simulink model "hdlcoder_counters_eml"  (R2026a)
settings: Solver=FixedStepDiscrete  StopTime=15  FixedStep=1
settings Model: Creator=The MathWorks, Inc.  LastModifiedBy=The MathWorks, Inc.
settings OptimizationCC: ConditionallyExecuteInputs=off  InitFltsAndDblsToZero=on
settings DebuggingCC: AlgebraicLoopMsg=error  SaveWithParameterizedLinksMsg=none  UnderspecifiedInitializationDetection=Classic  MultiTaskDSMMsg=warning  MultiTaskCondExecSysMsg=none  SingleTaskRateTransMsg=error
settings HardwareCC: ProdHWDeviceType=Specified
settings GRTTargetCC: TargetFcnLib=ansi_tfl_tmw.mat  CombineOutputUpdateFcns=off  GRTInterface=on

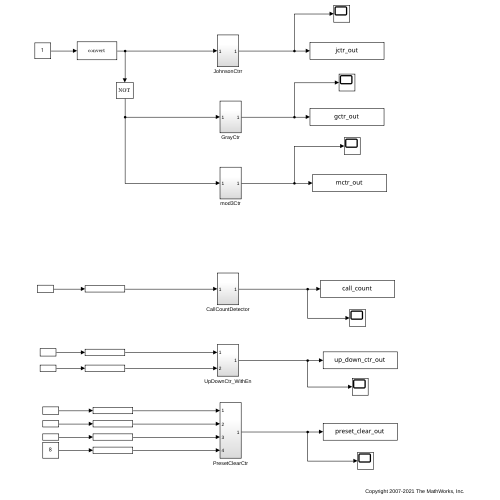
[thumbnail: Simulink's stored preview of the top-level diagram]
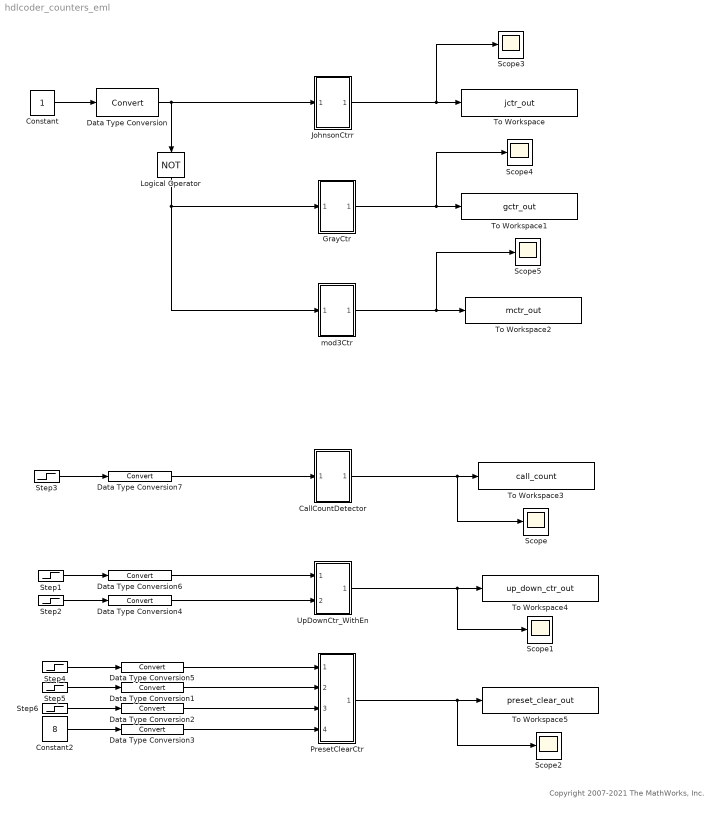
== system hdlcoder_counters_eml ==
  note: Copyright 2007-2021 The MathWorks, Inc.
  CallCountDetector : Subsystem
  Constant : Constant  SampleTime=1
  Constant2 : Constant  Value=8  SampleTime=1
  Data Type Conversion{,1..7} (8 alike) : DataTypeConversion  SaturateOnIntegerOverflow=off  RndMeth=Floor
  GrayCtr : Subsystem
  JohnsonCtrr : Subsystem
  Logical Operator : Logic  Operator=NOT  AllPortsSameDT=off  OutDataTypeStr=boolean
  PresetClearCtr : Subsystem
  Scope{,1..5} (6 alike) : Scope
      Scope2 settings: DataLoggingVariableName=ScopeData2
      Scope3 settings: DataLoggingVariableName=ScopeData3
      Scope4 settings: DataLoggingVariableName=ScopeData4
      Scope5 settings: DataLoggingVariableName=ScopeData5
  Step1 : Step  Time=3  SampleTime=1
  Step2 : Step  Time=7  SampleTime=1
  Step3 : Step  Time=3  SampleTime=1
  Step4 : Step  Time=7  SampleTime=1
  Step5 : Step  Time=2  SampleTime=1
  Step6 : Step  Time=4  SampleTime=1
  To Workspace : ToWorkspace  VariableName=jctr_out  SampleTime=-1
  To Workspace1 : ToWorkspace  VariableName=gctr_out  SampleTime=-1
  To Workspace2 : ToWorkspace  VariableName=mctr_out  SampleTime=-1
  To Workspace3 : ToWorkspace  VariableName=call_count  SampleTime=-1
  To Workspace4 : ToWorkspace  VariableName=up_down_ctr_out  SampleTime=-1
  To Workspace5 : ToWorkspace  VariableName=preset_clear_out  SampleTime=-1
  UpDownCtr_WithEn : Subsystem
  mod3Ctr : Subsystem
  wires:
  Constant/1 -> Data Type Conversion/1
  Data Type Conversion/1 -> Logical Operator/1, JohnsonCtrr/1(In1)
  Logical Operator/1 -> GrayCtr/1(In1), mod3Ctr/1(In1)
  JohnsonCtrr/1(Out1) -> To Workspace/1, Scope3/1
  GrayCtr/1(Out1) -> To Workspace1/1, Scope4/1
  mod3Ctr/1(Out1) -> To Workspace2/1, Scope5/1
  Step4/1 -> Data Type Conversion5/1
  Step5/1 -> Data Type Conversion1/1
  Step6/1 -> Data Type Conversion2/1
  Constant2/1 -> Data Type Conversion3/1
  Data Type Conversion5/1 -> PresetClearCtr/1(In1)
  Data Type Conversion1/1 -> PresetClearCtr/2(In2)
  Data Type Conversion2/1 -> PresetClearCtr/3(In3)
  Data Type Conversion3/1 -> PresetClearCtr/4(In4)
  CallCountDetector/1(Out1) -> To Workspace3/1, Scope/1
  UpDownCtr_WithEn/1(Out1) -> To Workspace4/1, Scope1/1
  PresetClearCtr/1(Out1) -> To Workspace5/1, Scope2/1
  Step1/1 -> Data Type Conversion6/1
  Step2/1 -> Data Type Conversion4/1
  Data Type Conversion6/1 -> UpDownCtr_WithEn/1(In1)
  Data Type Conversion4/1 -> UpDownCtr_WithEn/2(In2)
  Step3/1 -> Data Type Conversion7/1
  Data Type Conversion7/1 -> CallCountDetector/1(In1)

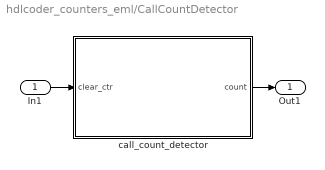
== system hdlcoder_counters_eml/CallCountDetector ==
  In1 : Inport
  call_count_detector : MATLAB Function  TreatAsAtomicUnit=on
  Out1 : Outport
  wires:
  In1/1 -> call_count_detector/1(clear_ctr)
  call_count_detector/1(count) -> Out1/1

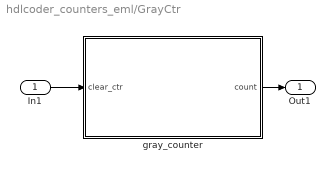
== system hdlcoder_counters_eml/GrayCtr ==
  In1 : Inport
  gray_counter : MATLAB Function  TreatAsAtomicUnit=on
  Out1 : Outport
  wires:
  In1/1 -> gray_counter/1(clear_ctr)
  gray_counter/1(count) -> Out1/1

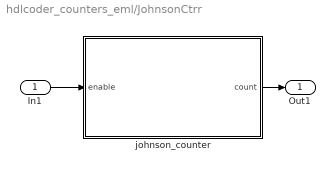
== system hdlcoder_counters_eml/JohnsonCtrr ==
  In1 : Inport
  johnson_counter : MATLAB Function  TreatAsAtomicUnit=on
  Out1 : Outport
  wires:
  In1/1 -> johnson_counter/1(enable)
  johnson_counter/1(count) -> Out1/1

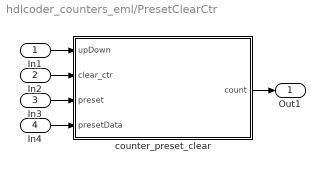
== system hdlcoder_counters_eml/PresetClearCtr ==
  In1 : Inport
  In2 : Inport  Port=2
  In3 : Inport  Port=3
  In4 : Inport  Port=4
  counter_preset_clear : MATLAB Function  TreatAsAtomicUnit=on
  Out1 : Outport
  wires:
  In1/1 -> counter_preset_clear/1(upDown)
  In2/1 -> counter_preset_clear/2(clear_ctr)
  counter_preset_clear/1(count) -> Out1/1
  In3/1 -> counter_preset_clear/3(preset)
  In4/1 -> counter_preset_clear/4(presetData)

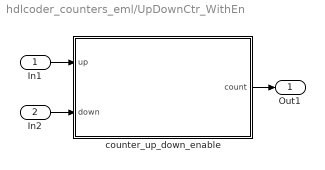
== system hdlcoder_counters_eml/UpDownCtr_WithEn ==
  In1 : Inport
  In2 : Inport  Port=2
  counter_up_down_enable : MATLAB Function  TreatAsAtomicUnit=on
  Out1 : Outport
  wires:
  In1/1 -> counter_up_down_enable/1(up)
  counter_up_down_enable/1(count) -> Out1/1
  In2/1 -> counter_up_down_enable/2(down)

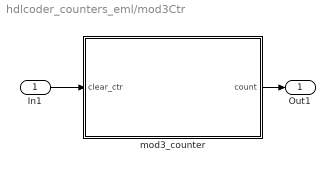
== system hdlcoder_counters_eml/mod3Ctr ==
  In1 : Inport
  mod3_counter : MATLAB Function  TreatAsAtomicUnit=on
  Out1 : Outport
  wires:
  In1/1 -> mod3_counter/1(clear_ctr)
  mod3_counter/1(count) -> Out1/1

== matlab function hdlcoder_counters_eml/PresetClearCtr/counter_preset_clear ==
  settings: fimath=|
      | fimath(...
      | 'RoundMode', 'floor',...
      | 'OverflowMode', 'saturate',...
      | 'ProductMode', 'FullPrecision', 'ProductWordLength', 32,...
      | 'SumMode', 'FullPrecision', 'SumWordLength', 32,...
      | 'CastBeforeSum', true)
  data: upDown input boolean; clear_ctr input boolean; preset input boolean; presetData input fixdt(0,4,0); count output fixdt(0,4,0) size=1
function count  = fcn(upDown, clear_ctr, preset, presetData)

% Up/down with synchronous preset and clear.
% With result_fm 'OverflowMode' set to saturate, this counter won't
% roll over.  Set to 'wrap' if rolling over is desirable.

result_nt = numerictype(0,4,0);
result_fm = fimath('OverflowMode', 'saturate', 'RoundMode', 'floor');

persistent count_reg;
if isempty(count_reg)
    count_reg = fi(0, result_nt, result_fm);
end

count = count_reg;

if clear_ctr
    count_reg = fi(0, result_nt, result_fm);
elseif preset
    count_reg = presetData;
elseif upDown
    inc = count_reg + fi(1, result_nt, result_fm);
    count_reg = fi(inc, result_nt, result_fm);
else
    dec = count_reg - fi(1, result_nt, result_fm);
    count_reg = fi(dec, result_nt, result_fm);
end

== matlab function hdlcoder_counters_eml/GrayCtr/gray_counter ==
  settings: sampleTime=.1
  settings: fimath=|
      | fimath(...
      | 'RoundMode', 'floor',...
      | 'OverflowMode', 'wrap',...
      | 'ProductMode', 'FullPrecision', 'ProductWordLength', 32,...
      | 'SumMode', 'FullPrecision', 'SumWordLength', 32,...
      | 'CastBeforeSum', true)
  data: clear_ctr input boolean; count output fixdt(0,4,0) size=1
function count = fcn(clear_ctr)

% A gray counter is a binary counter with the following conversion logic:

% 1. the first gray bit (msb) is same as first binary bit
% 2. the second gray bit is determined by xoring the second binary with the first binary bit and so on;
%    that is each pair of adjacent bits are xor'ed to get the next gray bit.
%
% This counter is configured to rollover.  Set result_fm to 'saturate'
% if rollver is not desirable.

result_nt = numerictype(0,4,0);
result_fm = fimath('OverflowMode', 'wrap', 'RoundMode', 'floor');

persistent bin_count;
if isempty(bin_count)
    bin_count = fi(0, result_nt, result_fm);
end

persistent gray_count;
if isempty(gray_count)
    gray_count = fi(0, result_nt, result_fm); %#ok<NASGU>
end

count = gray_count;

if clear_ctr
    bin_count =  fi(0, result_nt, result_fm);
    gray_count =  fi(0, result_nt, result_fm);
else
    inc = bin_count + fi(1, result_nt, result_fm);
    bin_count = fi(inc, result_nt, result_fm);

    gray_count = bitshift(bin_count, -1);
    gray_count = bitxor( gray_count, bin_count );
end

== matlab function hdlcoder_counters_eml/CallCountDetector/call_count_detector ==
  settings: fimath=|
      | fimath(...
      | 'RoundMode', 'floor',...
      | 'OverflowMode', 'wrap',...
      | 'ProductMode', 'FullPrecision', 'ProductWordLength', 32,...
      | 'SumMode', 'FullPrecision', 'SumWordLength', 32,...
      | 'CastBeforeSum', true)
  data: clear_ctr input boolean; count output fixdt(0,4,0) size=1
function count  = fcn(clear_ctr)

% A counter with synchronous clear, that counts how many times
% this block is called.
% 'count' saturates if called more than 15 times.
% Set 'OverflowMode' of result_fm to 'wrap' if you want the counter
% to roll over.

result_nt = numerictype(0,4,0);
result_fm = fimath('OverflowMode', 'saturate', 'RoundMode', 'floor');

persistent count_reg;
if isempty(count_reg)
    count_reg = fi(0, result_nt, result_fm);
end

count = count_reg;

if clear_ctr
    count_reg = fi(0, result_nt, result_fm);
else    
    inc = count_reg + fi(1, result_nt, result_fm);
    count_reg = fi(inc, result_nt, result_fm);
end

== matlab function hdlcoder_counters_eml/JohnsonCtrr/johnson_counter ==
  settings: fimath=|
      | fimath(...
      | 'RoundMode', 'floor',...
      | 'OverflowMode', 'saturate',...
      | 'ProductMode', 'FullPrecision', 'ProductWordLength', 32,...
      | 'SumMode', 'FullPrecision', 'SumWordLength', 32,...
      | 'CastBeforeSum', true)
  data: enable input boolean; count output fixdt(0,4,0) size=1
function count = fcn(enable)

% A johnson counter is a circular shift register that feeds the LSB with
% the inverted MSB.  It generates a pattern like
% 0000
% 0001
% 0011
% 0111
% 1111
% 1110
% 1100
% 1000
% 0000
% 0001

% This counter is configured to rollover.  If this is not desirable,
% set result_fm 'OverflowMode' to 'saturate'.

result_nt = numerictype(0,4,0);
result_fm = fimath('OverflowMode', 'wrap', 'RoundMode', 'floor');

persistent count_reg;

if isempty(count_reg)
    count_reg = fi(0, result_nt, result_fm);
end

% Assign the output even when we're not enabled.
count = count_reg;

if enable
   oldmsb = getmsb(count_reg);
   count_reg = bitsll(count_reg, 1);   
   count_reg = bitset(count_reg, 1, ~uint8(oldmsb));
end

== matlab function hdlcoder_counters_eml/mod3Ctr/mod3_counter ==
  settings: fimath=|
      | fimath(...
      | 'RoundMode', 'floor',...
      | 'OverflowMode', 'saturate',...
      | 'ProductMode', 'FullPrecision', 'ProductWordLength', 32,...
      | 'SumMode', 'FullPrecision', 'SumWordLength', 32,...
      | 'CastBeforeSum', true)
  data: clear_ctr input boolean; count output size=1
function count = fcn(clear_ctr)

% Count 0, 1, 2, 0, 1, 2

% This counter is configured to rollover.  If this is
% not desirable set result_fm 'OverflowMode' to 'saturate'.

result_nt = numerictype(0,3,0);
result_fm = fimath('OverflowMode', 'wrap', 'RoundMode', 'floor');

persistent count_reg;
if isempty(count_reg)
    count_reg = fi(0, result_nt, result_fm);
end

count = count_reg;

if clear_ctr
    count_reg = fi(0, result_nt, result_fm);
else
    t = fi(count_reg + 1, result_nt, result_fm);

    if (t <= fi(7, 0, 3, 0))
        count_reg = fi(t, result_nt, result_fm);
    else
        count_reg = fi(0, result_nt, result_fm);
    end    
end

== matlab function hdlcoder_counters_eml/UpDownCtr_WithEn/counter_up_down_enable ==
  settings: fimath=|
      | fimath(...
      | 'RoundMode', 'floor',...
      | 'OverflowMode', 'wrap',...
      | 'ProductMode', 'FullPrecision', 'ProductWordLength', 32,...
      | 'SumMode', 'FullPrecision', 'SumWordLength', 32,...
      | 'CastBeforeSum', true)
  data: count output fixdt(0,4,0) size=1; up input boolean; down input boolean
function count = fcn(up, down)

% synchronous up down counter
% If "up" is set, it counts up.
% Else, if "down" is set, it counts down
% If neither is set it's disabled.

result_nt = numerictype(0,4,0);

% With "saturate" set this counter willnever rollover.  To make it
% rollover, set the 'OverflowMode' to 'wrap'.
result_fm = fimath('OverflowMode', 'saturate', 'RoundMode', 'floor');

persistent count_reg;
if isempty(count_reg)
    count_reg = fi(0, result_nt, result_fm);
end

count = count_reg;

if up
    inc = count_reg + fi(1, result_nt, result_fm);
    count_reg = fi(inc, result_nt, result_fm);
elseif down
    dec = count_reg - fi(1, result_nt, result_fm);
    count_reg = fi(dec, result_nt, result_fm);
end
